simulink model "Engine_Component_harness_model"  (R2023a)
settings: Solver=daessc  StartTime=0.0  StopTime=30  RelTol=1e-3  AbsTol=1e-3
PreLoadFcn:
  | Engine_Component_harness_setup
libraries: fl_lib x11, nesl_utility x6, sdl_lib x2
settings Model: Creator=isaacito  LastModifiedBy=isaacito
settings OptimizationCC: ReuseModelBlockBuffer=off
settings ModelReferenceCC: EnableRefExpFcnMdlSchedulingChecks=on
settings SimscapeCC: SimscapeLogType=all  SimscapeLogSimulationStatistics=on  SimscapeLogLimitData=off

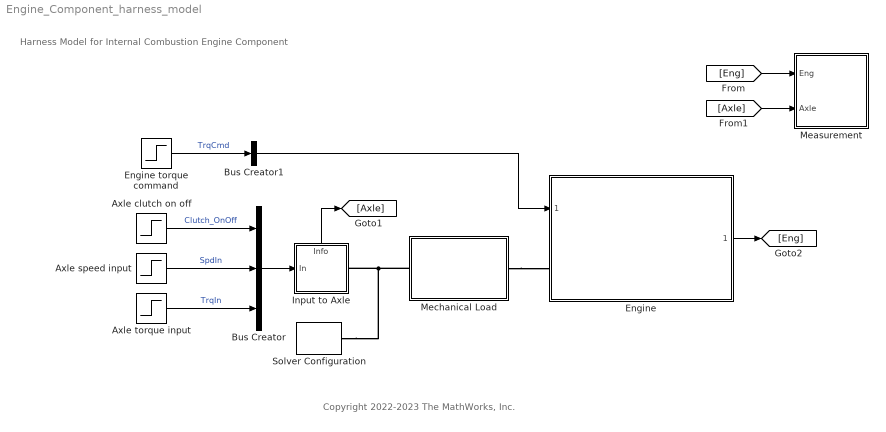
== system Engine_Component_harness_model ==
  note: Copyright 2022-2023 The MathWorks, Inc.
  note: Harness Model for Internal Combustion Engine Component
  Axle clutch on off : Step  After=0  SampleTime=0
  Axle speed input : Step  After=0  SampleTime=0
  Axle torque input : Step  Time=20  After=20  SampleTime=0
  Bus Creator : BusCreator  Inputs=3
  Bus Creator1 : BusCreator  Inputs=1
  Engine : Subsystem  ReferencedSubsystem=Engine_refsub_Basic
  Engine torque command : Step  Time=10  Before=40  After=100  SampleTime=0
  Input to Axle : Subsystem
      settings: PortSchema="{\"entries\":[{\"content\":{\"sides\":[{\"content\":{\"connectorIds\":[\"In1\"]},\"type\":\"ConnectorPlacement.EquallySpacedRectSide\",\"uuid\":\"17ecda4f-ad99-4587-a38d-a324d7486455\"},{\"content\":{\"connectorIds\":[\"RConn1\"],\"side\":\"RIGHT\"},\"type\":\"ConnectorPlacement.EquallySpacedRectSide\",\"uuid\":\"02def29b-e53d-45c2-af98-8005350a1631\"},{\"content\":{\"connectorIds\":[\"Out1\"],\"side\":\"TOP\"},\"type\":\"ConnectorPlacement.EquallySpacedRectSide\",\"uuid\":\"2d06855e-5bd1-4c4c-a72f-3146430204d1\"}]},\"type\":\"ConnectorPlacement.EquallySpacedConnector\",\"uuid\":\"a8d07ca5-35bb-4517-a87a-8359777d2cb9\"}],\"packageUris\":[\"http://schema.mathworks.com/mf0/Connector/R2020b\"],\"version\":\"1.0\"}"
  Measurement : Subsystem
  Mechanical Load : Subsystem
  Solver Configuration : nesl_utility/Solver Configuration  PhysicalDomain=network_engine_domain  SubClassName=solver  LeftPortType=input  RightPortType=generic  Tones=[]  Harmonics=[]  SimulateNoise=off  Profile=off  UseLocalSampling=off  EnableSwitchedLinearOptims=on  FrequencyDomain=off  UseCCode=off  RelTol=0.001  AbsTol=0.001  MinStep=1e-09  ToWorkspace=off  RevertToSquareIcSolve=off  NumHomotopyIterations=100  PhasorMode=off  PhasorModeNumHarmonics=1  ConsistencySolver=NEWTON_FTOL  IndexReductionMethod=DerivativeReplacement  DoDC=off  ResidualTolerance=1e-09  ConsistencyTolSource=GLOBAL  ConsistencyAbsTol=0.001  ConsistencyRelTol=0.001  ConsistencyTolFactor=0.001  UseLocalSolver=off  LocalSolverChoice=NE_BACKWARD_EULER_ADVANCER  ResolveIndetEquations=on  FunctionEvalNumThread=1  LocalSolverSampleTime=0.001  DoFixedCost=off  MaxNonlinIter=3  MaxModeIter=2  ComputeImpulses=off  ImpulseIterations=2  LinearAlgebra=auto  LinearAlgebraNumThread=0  EquationFormulation=NE_TIME_EF  DelaysMemoryBudget=1024  AutomaticFiltering=on  FilteringTimeConstant=0.001  PartitionStorageMethod=AS_NEEDED  PartitionMemoryBudget=1024  PartitionMethod=ROBUST
      settings: AttributesFormatString=Local solver: %<UseLocalSolver>
  wires:
  [Eng] -> Measurement/1(Eng)
  Axle clutch on off/1 -> Bus Creator/1  "Clutch_OnOff"
  Axle speed input/1 -> Bus Creator/2  "SpdIn"
  Axle torque input/1 -> Bus Creator/3  "TrqIn"
  Bus Creator/1 -> Input to Axle/1(In)
  Input to Axle/1(Info) -> [Axle]
  [Axle] -> Measurement/2(Axle)
  Engine/1 -> [Eng]
  Engine torque command/1 -> Bus Creator1/1  "TrqCmd"
  Bus Creator1/1 -> Engine/1
  connections:
  Mechanical Load/LConn1 -- Solver Configuration/RConn1 -- Input to Axle/RConn1
  Mechanical Load/RConn1 -- Engine/LConn1

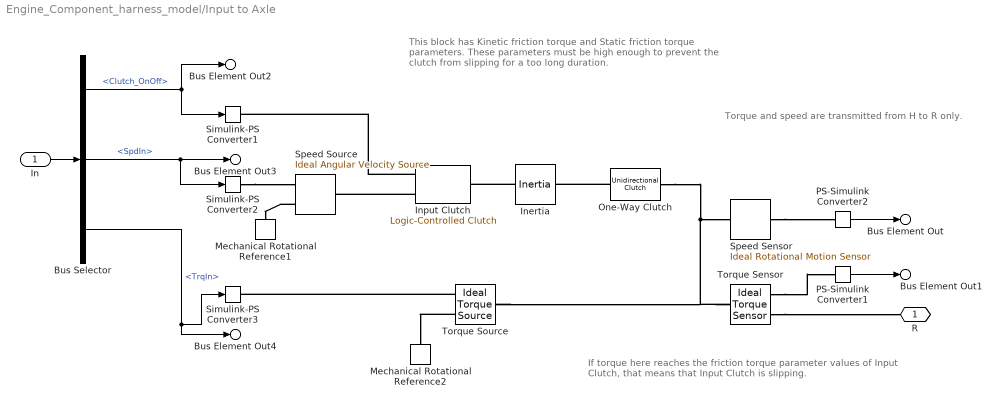
== system Engine_Component_harness_model/Input to Axle ==
  note: Torque and speed are transmitted
      | from H to R only.
  note: This block has Kinetic friction torque and
      | Static friction torque parameters.
      | These parameters must be high enough
      | to prevent the clutch from slipping
      | for a too long duration.
  note: If torque here reaches the friction torque
      | parameter values of Input Clutch,
      | that means that Input Clutch is slipping.
  In : Inport
      settings: AttributesFormatString=%<Unit>
  Bus Selector : BusSelector  OutputSignals=Clutch_OnOff,SpdIn,TrqIn
  Inertia : fl_lib/Mechanical/Rotational Elements/Inertia  inertia=0.001 kg*m^2  num_ports=foundation.enum.numPorts2.two  w_specify=on  w_priority=None  w=0 rad/s  w_nominal_specify=off  w_nominal_unit=rad/s  w_nominal_value=1  t_specify=off  t_priority=None  t=0 N*m  t_nominal_specify=off  t_nominal_unit=N*m  t_nominal_value=1
      settings: InternalSimscapePortConfiguration="{\"Bottom\":[],\"Left\":[{\"id\":\"I\",\"label\":\"\",\"type\":\"foundation.mechanical.rotational.rotational\"}],\"Right\":[{\"id\":\"J\",\"label\":\"\",\"type\":\"foundation.mechanical.rotational.rotational\"}],\"Top\":[]}"
  Input Clutch : sdl_lib/Clutches/Logic-Controlled Clutch  transition_model=sdl.enum.transitionModel.instant  transition_time_constant=0.1 s  t_friction=900 kN*m  t_locked=900 kN*m  w_tol=0.001 rad/s  initial_state_locked=sdl.enum.initial_lock.unlocked
      settings: AttributesFormatString=%<initial_state_locked>  InternalSimscapePortConfiguration="{\"Bottom\":[],\"Left\":[{\"id\":\"E\",\"label\":\"E\",\"type\":\"input\"},{\"id\":\"B\",\"label\":\"B\",\"type\":\"foundation.mechanical.rotational.rotational\"}],\"Right\":[{\"id\":\"F\",\"label\":\"F\",\"type\":\"foundation.mechanical.rotational.rotational\"}],\"Top\":[]}"
  Mechanical Rotational Reference1 : fl_lib/Mechanical/Rotational Elements/Mechanical Rotational Reference
  Mechanical Rotational Reference2 : fl_lib/Mechanical/Rotational Elements/Mechanical Rotational Reference
  One-Way Clutch : sdl_lib/Clutches/Unidirectional Clutch  transmission_direction=sdl.enum.hubRingDirection.positive  initial_state_locked=sdl.enum.initial_lock.unlocked
      settings: InternalSimscapePortConfiguration="{\"Bottom\":[],\"Left\":[{\"id\":\"H\",\"label\":\"H\",\"type\":\"foundation.mechanical.rotational.rotational\"}],\"Right\":[{\"id\":\"R\",\"label\":\"R\",\"type\":\"foundation.mechanical.rotational.rotational\"}],\"Top\":[]}"
  PS-Simulink Converter1 : nesl_utility/PS-Simulink Converter  PhysicalDomain=network_engine_domain  SubClassName=ps_output  LeftPortType=input  RightPortType=output  PseudoPeriodic=off  Frequencies=[]  VectorFormat=1-D array  Unit=N*m  AffineConversion=off
  PS-Simulink Converter2 : nesl_utility/PS-Simulink Converter  PhysicalDomain=network_engine_domain  SubClassName=ps_output  LeftPortType=input  RightPortType=output  PseudoPeriodic=off  Frequencies=[]  VectorFormat=1-D array  Unit=rpm  AffineConversion=off
  Simulink-PS Converter1 : nesl_utility/Simulink-PS Converter  PhysicalDomain=network_engine_domain  SubClassName=ps_input  LeftPortType=input  RightPortType=output  PseudoPeriodic=off  Frequencies=[]  NoiseDistribution=none  NoiseParameters=[]  Unit=1  AffineConversion=off  FilteringAndDerivatives=zero  SimscapeFilterOrder=1  InputFilterTimeConstant=0.001  UdotUserProvided=0
  Simulink-PS Converter2 : nesl_utility/Simulink-PS Converter  PhysicalDomain=network_engine_domain  SubClassName=ps_input  LeftPortType=input  RightPortType=output  PseudoPeriodic=off  Frequencies=[]  NoiseDistribution=none  NoiseParameters=[]  Unit=rpm  AffineConversion=off  FilteringAndDerivatives=filter  SimscapeFilterOrder=1  InputFilterTimeConstant=0.001  UdotUserProvided=0
  Simulink-PS Converter3 : nesl_utility/Simulink-PS Converter  PhysicalDomain=network_engine_domain  SubClassName=ps_input  LeftPortType=input  RightPortType=output  PseudoPeriodic=off  Frequencies=[]  NoiseDistribution=none  NoiseParameters=[]  Unit=N*m  AffineConversion=off  FilteringAndDerivatives=filter  SimscapeFilterOrder=1  InputFilterTimeConstant=0.001  UdotUserProvided=0
  Speed Sensor : fl_lib/Mechanical/Mechanical Sensors/Ideal Rotational Motion Sensor  reference=foundation.enum.MeasurementReference.absolute  acceleration_port=false  velocity_port=true  position_port=false  wrap_angle=simscape.enum.onoff.off  offset=0 rad
      settings: InternalSimscapePortConfiguration="{\"Bottom\":[],\"Left\":[{\"id\":\"R\",\"label\":\"R\",\"type\":\"foundation.mechanical.rotational.rotational\"}],\"Right\":[{\"id\":\"W\",\"label\":\"W\",\"type\":\"output\"}],\"Top\":[]}"
  Speed Source : fl_lib/Mechanical/Mechanical Sources/Ideal Angular Velocity Source
  Torque Sensor : fl_lib/Mechanical/Mechanical Sensors/Ideal Torque Sensor
  Torque Source : fl_lib/Mechanical/Mechanical Sources/Ideal Torque Source
  R : PMIOPort  Side=Right
  Bus Element Out : Outport  PortName=Info  Element=AxleSpd
  Bus Element Out1 : Outport  PortName=Info  Element=AxleTrq
  Bus Element Out2 : Outport  PortName=Info  Element=ClutchOnOff
  Bus Element Out3 : Outport  PortName=Info  Element=SpdIn
  Bus Element Out4 : Outport  PortName=Info  Element=TrqIn
  wires:
  PS-Simulink Converter2/1 -> Bus Element Out/1
  PS-Simulink Converter1/1 -> Bus Element Out1/1
  In/1 -> Bus Selector/1
  Bus Selector/1 -> Simulink-PS Converter1/1, Bus Element Out2/1  "<Clutch_OnOff>"
  Bus Selector/2 -> Simulink-PS Converter2/1, Bus Element Out3/1  "<SpdIn>"
  Bus Selector/3 -> Bus Element Out4/1, Simulink-PS Converter3/1  "<TrqIn>"
  connections:
  Torque Sensor/RConn2 -- PS-Simulink Converter1/LConn1
  One-Way Clutch/RConn1 -- Torque Sensor/LConn1 -- Torque Source/LConn1 -- Speed Sensor/LConn1
  Simulink-PS Converter2/RConn1 -- Speed Source/RConn1
  Speed Source/RConn2 -- Mechanical Rotational Reference1/LConn1
  Input Clutch/LConn2 -- Speed Source/LConn1
  Torque Sensor/RConn1 -- R/RConn1
  Input Clutch/LConn1 -- Simulink-PS Converter1/RConn1
  Speed Sensor/RConn1 -- PS-Simulink Converter2/LConn1
  Torque Source/RConn2 -- Mechanical Rotational Reference2/LConn1
  Torque Source/RConn1 -- Simulink-PS Converter3/RConn1
  One-Way Clutch/LConn1 -- Inertia/RConn1
  Inertia/LConn1 -- Input Clutch/RConn1

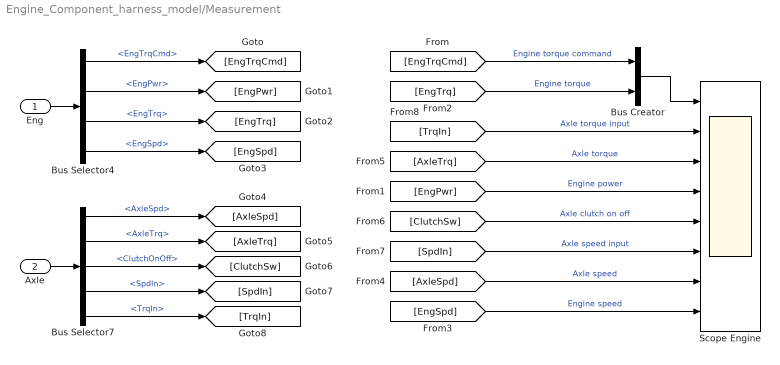
== system Engine_Component_harness_model/Measurement ==
  Eng : Inport
  Axle : Inport  Port=2
  Bus Creator : BusCreator  Inputs=2
  Bus Selector4 : BusSelector  OutputSignals=EngTrqCmd,EngPwr,EngTrq,EngSpd
  Bus Selector7 : BusSelector  OutputSignals=AxleSpd,AxleTrq,ClutchOnOff,SpdIn,TrqIn
  Scope Engine : Scope  NumInputPorts=8
  wires:
  Eng/1 -> Bus Selector4/1
  Axle/1 -> Bus Selector7/1
  Bus Selector7/1 -> [AxleSpd]  "<AxleSpd>"
  Bus Selector7/2 -> [AxleTrq]  "<AxleTrq>"
  Bus Selector4/1 -> [EngTrqCmd]  "<EngTrqCmd>"
  Bus Selector4/2 -> [EngPwr]  "<EngPwr>"
  Bus Selector4/3 -> [EngTrq]  "<EngTrq>"
  Bus Selector4/4 -> [EngSpd]  "<EngSpd>"
  Bus Selector7/3 -> [ClutchSw]  "<ClutchOnOff>"
  Bus Selector7/4 -> [SpdIn]  "<SpdIn>"
  Bus Selector7/5 -> [TrqIn]  "<TrqIn>"
  [EngTrqCmd] -> Bus Creator/1  "Engine torque command"
  [EngTrq] -> Bus Creator/2  "Engine torque"
  Bus Creator/1 -> Scope Engine/1
  [TrqIn] -> Scope Engine/2  "Axle torque input"
  [AxleTrq] -> Scope Engine/3  "Axle torque"
  [EngPwr] -> Scope Engine/4  "Engine power"
  [ClutchSw] -> Scope Engine/5  "Axle clutch on off"
  [SpdIn] -> Scope Engine/6  "Axle speed input"
  [AxleSpd] -> Scope Engine/7  "Axle speed"
  [EngSpd] -> Scope Engine/8  "Engine speed"

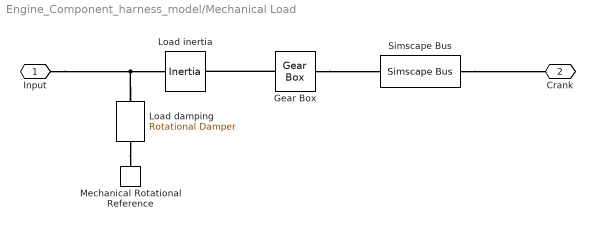
== system Engine_Component_harness_model/Mechanical Load ==
  Gear Box : fl_lib/Mechanical/Mechanisms/Gear Box  ratio=1  t_in_specify=off  t_in_priority=None  t_in=0 N*m  t_in_nominal_specify=off  t_in_nominal_unit=N*m  t_in_nominal_value=1  t_out_specify=off  t_out_priority=None  t_out=0 N*m  t_out_nominal_specify=off  t_out_nominal_unit=N*m  t_out_nominal_value=1
      settings: AttributesFormatString=Gear ratio: %<ratio>
  Load damping : fl_lib/Mechanical/Rotational Elements/Rotational Damper  D=0.001 m*N/rpm  w_specify=off  w_priority=None  w=0 rad/s  w_nominal_specify=off  w_nominal_unit=rad/s  w_nominal_value=1  t_specify=off  t_priority=None  t=0 N*m  t_nominal_specify=off  t_nominal_unit=N*m  t_nominal_value=1
      settings: AttributesFormatString=%<D> %<D_unit>
  Load inertia : fl_lib/Mechanical/Rotational Elements/Inertia  inertia=10*0.1^2 kg*m^2  num_ports=foundation.enum.numPorts2.two  w_specify=on  w_priority=High  w=initial.loadInertia_speed_rpm rpm  w_nominal_specify=off  w_nominal_unit=rad/s  w_nominal_value=1  t_specify=off  t_priority=None  t=0 N*m  t_nominal_specify=off  t_nominal_unit=N*m  t_nominal_value=1
      settings: InternalSimscapePortConfiguration="{\"Bottom\":[],\"Left\":[{\"id\":\"I\",\"label\":\"\",\"type\":\"foundation.mechanical.rotational.rotational\"}],\"Right\":[{\"id\":\"J\",\"label\":\"\",\"type\":\"foundation.mechanical.rotational.rotational\"}],\"Top\":[]}"
      settings: AttributesFormatString=|
      | %<w> [%<w_unit>]
      | Priority: %<w_priority>
      | %<inertia> %<inertia_unit>
  Mechanical Rotational Reference : fl_lib/Mechanical/Rotational Elements/Mechanical Rotational Reference
  Simscape Bus : SimscapeBus  HierarchyStrings=AngSpd  ConnectionType=Bus: Bus_Rotational
      settings: AttributesFormatString=%<ConnectionType>
  Input : PMIOPort  Side=Left
  Crank : PMIOPort  Port=2  Side=Right
  connections:
  Gear Box/RConn1 -- Load inertia/LConn1
  Load damping/RConn1 -- Mechanical Rotational Reference/LConn1
  Simscape Bus/RConn1 -- Crank/RConn1
  Gear Box/LConn1 -- Simscape Bus/LConn1
  Input/RConn1 -- Load damping/LConn1 -- Load inertia/RConn1
